simulink model "Simulink_ABS_Q4"  (R2026b)
settings: Solver=VariableStepAuto  StopTime=10  MaxStep=1e-3
InitFcn:
  | Code_ABS
values from neighbouring files (symbols this model uses):
  A = 4000    [Code_ABS.m]
  acc = -1/m    (= -0.001)    [Code_ABS.m]
  f_adh = 0.8    [Code_ABS.m]
  f_tab = [0 0.60 0.85 0.93 0.95 0.88 0.80 0.73 0.68 0.63 0.60]    [Code_ABS.m]
  gliss_tab = [0 0.05 0.10 0.15 0.20 0.30 0.40 0.50 0.60 0.80 1.00]    [Code_ABS.m]
  J = 0.5    [Code_ABS.m]
  k_tr = m*h/(2*L)    (= 116.666666667)    [Code_ABS.m]
  N0 = m*g0/4    (= 2452.5)    [Code_ABS.m]
  N_ar0 = m*g0*l_av/(2*L)    (= 2452.5)    [Code_ABS.m]
  N_av0 = m*g0*l_ar/(2*L)    (= 2452.5)    [Code_ABS.m]
  rRoue = 0.3    [Code_ABS.m]
  tau_a = 0.02    [Code_ABS.m]
  v0 = 27.77    [Code_ABS.m]
libraries: sl_discontinuities x2, simulink x2
settings Model: Creator=Tom  LastModifiedBy=Tom

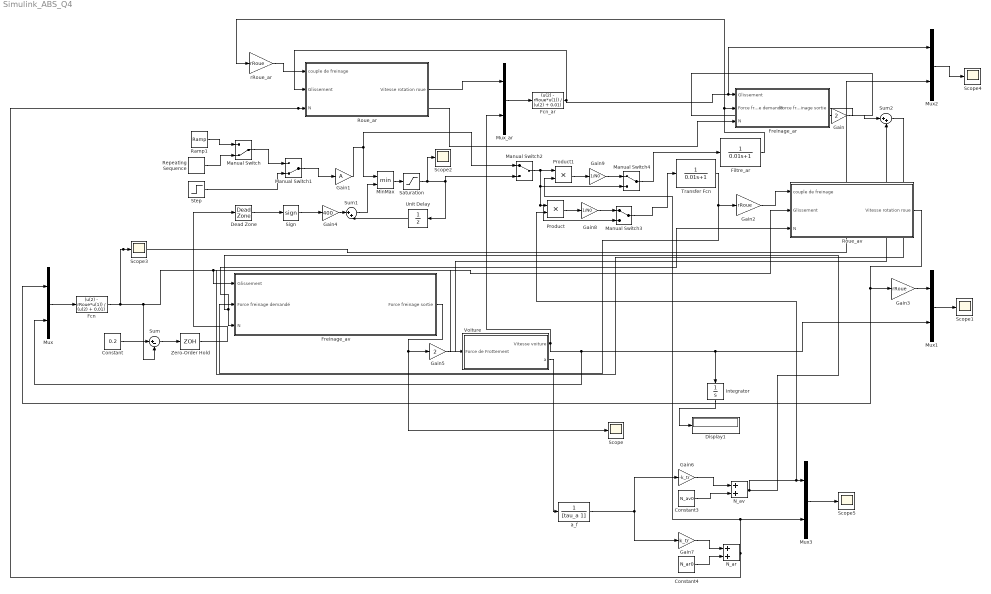
== system Simulink_ABS_Q4 ==
  Constant : Constant  Value=0.2
  Constant3 : Constant  Value=N_av0
  Constant4 : Constant  Value=N_ar0
  Dead Zone : DeadZone  LowerValue=-0.01  UpperValue=0.01
  Display1 : Display
  Fcn : Fcn  Expr=(u(2) - rRoue*u(1)) / (u(2) + 0.01)
  Fcn_ar : Fcn  Expr=(u(2) - rRoue*u(1)) / (u(2) + 0.01)
  Filtre_ar : TransferFcn  Denominator=[0.01 1]
  Freinage_ar : Subsystem
  Freinage_av : Subsystem
  Gain : Gain  Gain=2
  Gain1 : Gain  Gain=A
  Gain2 : Gain  Gain=rRoue
  Gain3 : Gain  Gain=rRoue
  Gain4 : Gain  Gain=400
  Gain5 : Gain  Gain=2
  Gain6 : Gain  Gain=-k_tr
  Gain7 : Gain  Gain=k_tr
  Gain8 : Gain  Gain=1/N0
  Gain9 : Gain  Gain=1/N0
  Integrator : Integrator
  Manual Switch : ManualSwitch  CurrentSetting=0
  Manual Switch1 : ManualSwitch  CurrentSetting=0
  Manual Switch2 : ManualSwitch
  Manual Switch3 : ManualSwitch
  Manual Switch4 : ManualSwitch
  MinMax : MinMax  Inputs=2
  Mux{,1..3} (4 alike) : Mux  Inputs=2
  Mux_ar : Mux  Inputs=2
  N_ar : Sum
  N_av : Sum
  Product : Product
  Product1 : Product
  Ramp1 : simulink/Sources/Ramp  slope=1000  start=0  InitialOutput=0
  Repeating Sequence : simulink/Sources/Repeating Sequence  rep_seq_t=[0 1 8 9 10]  rep_seq_y=[0 1 1 0 0]
  Roue_ar : Subsystem
  Roue_av : Subsystem
  Saturation : Saturate  UpperLimit=inf  LowerLimit=0
  Scope{,1..5} (6 alike) : Scope
      Scope settings: ActiveDisplayYMinimum=471.5  ActiveDisplayYMaximum=2471.5
      Scope1 settings: ActiveDisplayYMinimum=-3.4712499999999991  ActiveDisplayYMaximum=31.24125
      Scope2 settings: ActiveDisplayYMinimum=2388.1770780684733  ActiveDisplayYMaximum=2539.2393617203752  DataLoggingVariableName=ScopeData2
      Scope3 settings: ActiveDisplayYMinimum=0.11711730188145665  ActiveDisplayYMaximum=0.18650673751599733  DataLoggingVariableName=ScopeData3
      Scope4 settings: ActiveDisplayYMinimum=-0.12495414069391772  ActiveDisplayYMaximum=1.1245872662452596  DataLoggingVariableName=ScopeData4
      Scope5 settings: ActiveDisplayYMinimum=1376.9172468630957  ActiveDisplayYMaximum=3528.0827531369046  DataLoggingVariableName=ScopeData5
  Sign : Signum
  Step : Step  Time=0  SampleTime=0
  Sum : Sum  Inputs=|+-
  Sum1 : Sum  Inputs=|++
  Sum2 : Sum  Inputs=|++
  Transfer Fcn : TransferFcn  Denominator=[0.01 1]
  Unit Delay : UnitDelay  SampleTime=1e-4
  Voiture : Subsystem
  Zero-Order Hold : ZeroOrderHold  SampleTime=1e-4
  a_f : TransferFcn  Denominator=[tau_a 1]
  rRoue_ar : Gain  Gain=rRoue
  wires:
  Freinage_av/1(Force freinage sortie) -> Gain5/1, Scope/1
  Ramp1/1 -> Manual Switch/1
  Repeating Sequence/1 -> Manual Switch/2
  Step/1 -> Manual Switch1/2
  Manual Switch/1 -> Manual Switch1/1
  Manual Switch1/1 -> Gain1/1
  Gain1/1 -> Manual Switch2/1, MinMax/1
  Gain2/1 -> Roue_av/1(couple de freinage)
  Roue_av/1(Vitesse rotation roue) -> Gain3/1, Mux/1
  Mux/1 -> Fcn/1
  Fcn/1 -> Scope3/1, Mux2/2, Sum/2, Roue_av/2(Glissement), Freinage_av/1(Glissement)
  Voiture/1(Vitesse voiture) -> Mux1/2, Integrator/1, Mux/2, Mux_ar/2
  Integrator/1 -> Display1/1
  Mux1/1 -> Scope1/1
  Gain3/1 -> Mux1/1
  Transfer Fcn/1 -> Freinage_av/2(Force freinage demandé), Gain2/1
  Constant/1 -> Sum/1
  Zero-Order Hold/1 -> Dead Zone/1
  MinMax/1 -> Saturation/1
  Sum/1 -> Zero-Order Hold/1
  Sign/1 -> Gain4/1
  Gain4/1 -> Sum1/1
  Sum1/1 -> MinMax/2
  Saturation/1 -> Scope2/1, Unit Delay/1, Manual Switch2/2
  Unit Delay/1 -> Sum1/2
  Dead Zone/1 -> Sign/1
  N_av/1 -> Product/2, Mux3/1, Roue_av/3(N), Freinage_av/3(N)
  Roue_ar/1(Vitesse rotation roue) -> Mux_ar/1
  Mux_ar/1 -> Fcn_ar/1
  Fcn_ar/1 -> Roue_ar/2(Glissement), Mux2/1, Freinage_ar/1(Glissement)
  Gain5/1 -> Sum2/2
  Freinage_ar/1(Force freinage sortie) -> Gain/1
  Gain/1 -> Sum2/1
  Sum2/1 -> Voiture/1(Force de Frottement)
  Filtre_ar/1 -> rRoue_ar/1, Freinage_ar/2(Force freinage demandé)
  rRoue_ar/1 -> Roue_ar/1(couple de freinage)
  Mux2/1 -> Scope4/1
  Voiture/2(a) -> a_f/1
  a_f/1 -> Gain7/1, Gain6/1
  Gain7/1 -> N_ar/1
  Constant3/1 -> N_av/2
  Gain6/1 -> N_av/1
  Constant4/1 -> N_ar/2
  N_ar/1 -> Freinage_ar/3(N), Roue_ar/3(N), Mux3/2, Product1/2
  Mux3/1 -> Scope5/1
  Manual Switch2/1 -> Manual Switch3/2, Product/1, Manual Switch4/2, Product1/1
  Product/1 -> Gain8/1
  Gain8/1 -> Manual Switch3/1
  Manual Switch3/1 -> Transfer Fcn/1
  Product1/1 -> Gain9/1
  Gain9/1 -> Manual Switch4/1
  Manual Switch4/1 -> Filtre_ar/1

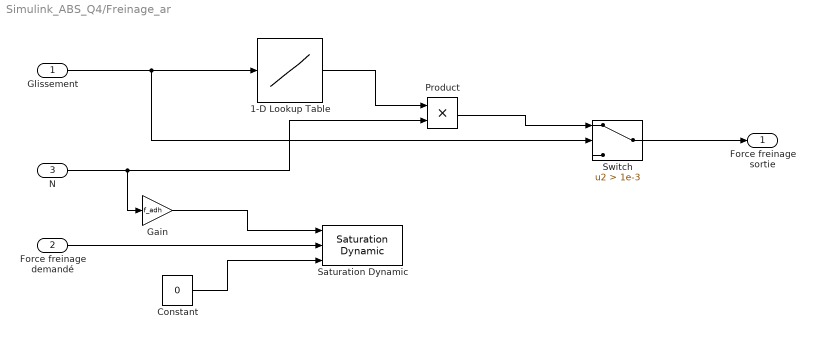
== system Simulink_ABS_Q4/Freinage_ar ==
  Glissement : Inport
  Force freinage demandé : Inport  Port=2
  N : Inport  Port=3
  1-D Lookup Table : Lookup_n-D  NumberOfTableDimensions=1  BreakpointsForDimension1=gliss_tab  Table=f_tab  InternalRulePriority=Speed  RndMeth=Simplest
  Constant : Constant  Value=0
  Gain : Gain  Gain=f_adh
  Product : Product
  Saturation Dynamic : sl_discontinuities/Saturation Dynamic  OutMin=[]  OutMax=[]  OutDataTypeStr=Inherit: Same as second input  OutDataType=fixdt(1, 16)  OutScaling=2^-10  DoSatur=off
      settings: LibrarySourceBlock=|
      | simulink/Discontinuities/Saturation
      | Dynamic
  Switch : Switch  Criteria=u2 > Threshold  Threshold=1e-3  SaturateOnIntegerOverflow=off  InputSameDT=off
  Force freinage sortie : Outport
  wires:
  1-D Lookup Table/1 -> Product/1
  Glissement/1 -> 1-D Lookup Table/1, Switch/2
  Switch/1 -> Force freinage sortie/1
  N/1 -> Gain/1, Product/2
  Product/1 -> Switch/1
  Force freinage demandé/1 -> Saturation Dynamic/2
  Gain/1 -> Saturation Dynamic/1
  Constant/1 -> Saturation Dynamic/3

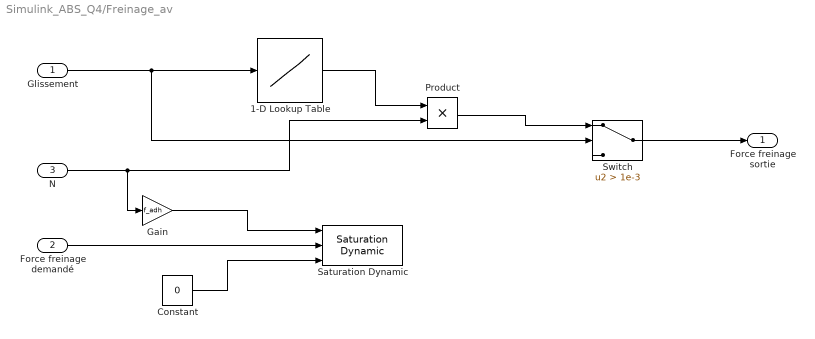
== system Simulink_ABS_Q4/Freinage_av ==
  Glissement : Inport
  Force freinage demandé : Inport  Port=2
  N : Inport  Port=3
  1-D Lookup Table : Lookup_n-D  NumberOfTableDimensions=1  BreakpointsForDimension1=gliss_tab  Table=f_tab  InternalRulePriority=Speed  RndMeth=Simplest
  Constant : Constant  Value=0
  Gain : Gain  Gain=f_adh
  Product : Product
  Saturation Dynamic : sl_discontinuities/Saturation Dynamic  OutMin=[]  OutMax=[]  OutDataTypeStr=Inherit: Same as second input  OutDataType=fixdt(1, 16)  OutScaling=2^-10  DoSatur=off
      settings: LibrarySourceBlock=|
      | simulink/Discontinuities/Saturation
      | Dynamic
  Switch : Switch  Criteria=u2 > Threshold  Threshold=1e-3  SaturateOnIntegerOverflow=off  InputSameDT=off
  Force freinage sortie : Outport
  wires:
  1-D Lookup Table/1 -> Product/1
  Glissement/1 -> 1-D Lookup Table/1, Switch/2
  Switch/1 -> Force freinage sortie/1
  N/1 -> Gain/1, Product/2
  Product/1 -> Switch/1
  Force freinage demandé/1 -> Saturation Dynamic/2
  Gain/1 -> Saturation Dynamic/1
  Constant/1 -> Saturation Dynamic/3

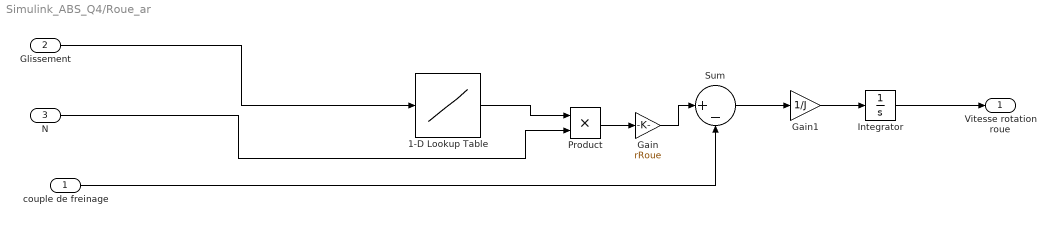
== system Simulink_ABS_Q4/Roue_ar ==
  couple de freinage : Inport
  Glissement : Inport  Port=2
  N : Inport  Port=3
  1-D Lookup Table : Lookup_n-D  NumberOfTableDimensions=1  BreakpointsForDimension1=gliss_tab  Table=f_tab  InternalRulePriority=Speed  RndMeth=Simplest
  Gain : Gain  Gain=rRoue
  Gain1 : Gain  Gain=1/J
  Integrator : Integrator  InitialCondition=v0/rRoue  LimitOutput=on  LowerSaturationLimit=0
  Product : Product
  Sum : Sum  Inputs=|+-
  Vitesse rotation roue : Outport
  wires:
  1-D Lookup Table/1 -> Product/1
  Gain1/1 -> Integrator/1
  Glissement/1 -> 1-D Lookup Table/1
  Sum/1 -> Gain1/1
  Integrator/1 -> Vitesse rotation roue/1
  couple de freinage/1 -> Sum/2
  N/1 -> Product/2
  Product/1 -> Gain/1
  Gain/1 -> Sum/1

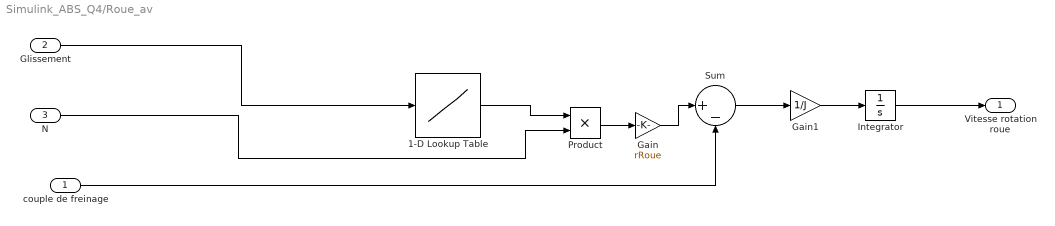
== system Simulink_ABS_Q4/Roue_av ==
  couple de freinage : Inport
  Glissement : Inport  Port=2
  N : Inport  Port=3
  1-D Lookup Table : Lookup_n-D  NumberOfTableDimensions=1  BreakpointsForDimension1=gliss_tab  Table=f_tab  InternalRulePriority=Speed  RndMeth=Simplest
  Gain : Gain  Gain=rRoue
  Gain1 : Gain  Gain=1/J
  Integrator : Integrator  InitialCondition=v0/rRoue  LimitOutput=on  LowerSaturationLimit=0
  Product : Product
  Sum : Sum  Inputs=|+-
  Vitesse rotation roue : Outport
  wires:
  1-D Lookup Table/1 -> Product/1
  Gain1/1 -> Integrator/1
  Glissement/1 -> 1-D Lookup Table/1
  Sum/1 -> Gain1/1
  Integrator/1 -> Vitesse rotation roue/1
  couple de freinage/1 -> Sum/2
  N/1 -> Product/2
  Product/1 -> Gain/1
  Gain/1 -> Sum/1

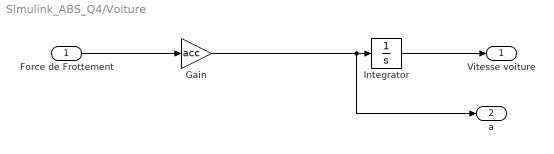
== system Simulink_ABS_Q4/Voiture ==
  Force de Frottement : Inport
  Gain : Gain  Gain=acc
  Integrator : Integrator  InitialCondition=v0  LimitOutput=on  LowerSaturationLimit=0
  Vitesse voiture : Outport
  a : Outport  Port=2
  wires:
  Gain/1 -> a/1, Integrator/1
  Force de Frottement/1 -> Gain/1
  Integrator/1 -> Vitesse voiture/1
